simulink model "communication_codegen_check"  (R2024b)
settings: Solver=FixedStepDiscrete  StartTime=0.0  StopTime=0.1  FixedStep=0.001  RelTol=1e-3
settings Model: Creator=Administrator  LastModifiedBy=Administrator
settings OptimizationCC: EnhancedBackFolding=on  PassReuseOutputArgsAs=Individual arguments  ZeroExternalMemoryAtStartup=off  ZeroInternalMemoryAtStartup=off  MaxStackSize=64  OptimizeBlockOrder=speed  DifferentSizesBufferReuse=on  OptimizationCustomize=off  EfficientTunableParamExpr=on
settings DebuggingCC: ParameterTunabilityLossMsg=error
settings HardwareCC: ProdBitPerLong=64  ProdHWDeviceType=Intel->x86-64 (Linux 64)
settings SFSimCC: MATLABDynamicMemAlloc=off
settings RTWCC: Description=Embedded Coder  SystemTargetFile=ert.tlc  HardwareBoard=SimRT  TLCOptions="-aInlineSetEventsForThisBaseRateFcn=TLC_FALSE -aSuppressMultiTaskScheduler=TLC_FALSE  -aRateBasedStepFcn=0"  TemplateMakefile=ert_default_tmf  Toolchain=X280 portable-linux-toolchain
settings CodeAppCC: ForceParamTrailComments=on  IgnoreCustomStorageClasses=off  OperatorAnnotations=on  SimulinkDataObjDesc=on  SFDataObjDesc=on  InsertBlockDesc=on
settings ERTTargetCC: ExtMode=on  ExtModeTransport=2  ExtModeStaticAlloc=on  ExtModeMexFile=ext_xcp  ExtModeIntrfLevel=Level2 - Open  InlinedParameterPlacement=Hierarchical

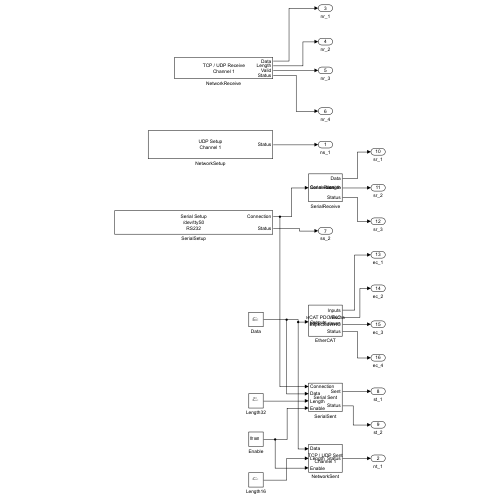
[thumbnail: Simulink's stored preview of the top-level diagram]
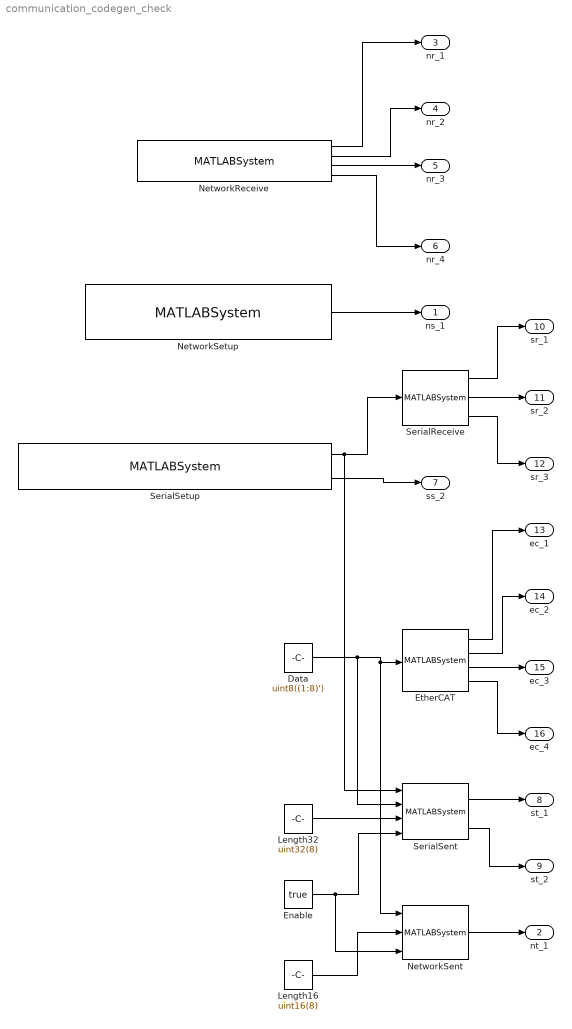
== system communication_codegen_check ==
  Data : Constant  Value=uint8((1:8)')
  Enable : Constant  Value=true
  EtherCAT : MATLABSystem  System=x280linux.ethercat.EtherCATExchange  Interface=eth1  ExpectedSlaves=1  OutputBytes=8  InputBytes=8  ReceiveTimeoutUs=500  SampleTime=0.001
      mask Type: x280linux.ethercat.EtherCATExchange
      mask Display:
      | disp(['EtherCAT PDO Exchange' char(10) 'eth1 / 1 slaves']);
      | port_label('input',1,'Outputs');
      | port_label('output',1,'Inputs');
      | port_label('output',2,'WKC');
      | port_label('output',3,'ExpectedWKC');
      | port_label('output',4,'Status');
  Length16 : Constant  Value=uint16(8)
  Length32 : Constant  Value=uint32(8)
  NetworkReceive : MATLABSystem  System=x280linux.net.TCPReceive  Channel=1  BufferSize=8  SampleTime=0.001
      mask Type: x280linux.net.TCPReceive
      mask Display:
      | disp(['TCP / UDP Receive' char(10) 'Channel 1']);
      | port_label('output',1,'Data');
      | port_label('output',2,'Length');
      | port_label('output',3,'Valid');
      | port_label('output',4,'Status');
  NetworkSent : MATLABSystem  System=x280linux.net.TCPSent  Channel=1
      mask Type: x280linux.net.TCPSent
      mask Display:
      | disp(['TCP / UDP Sent' char(10) 'Channel 1']);
      | port_label('input',1,'Data');
      | port_label('input',2,'Length');
      | port_label('input',3,'Enable');
      | port_label('output',1,'Status');
  NetworkSetup : MATLABSystem  System=x280linux.net.TCPSetup  Channel=1  Protocol=UDP  Role=Client  LocalAddress=0.0.0.0  LocalPort=45190  RemoteAddress=127.0.0.1  RemotePort=45191  SampleTime=0.001
      mask Type: x280linux.net.TCPSetup
      mask Display:
      | disp(['UDP Setup' char(10) 'Channel 1']);
      | port_label('output',1,'Status');
  SerialReceive : MATLABSystem  System=x280linux.serial.SerialReceive  BufferSize=8
      mask Type: x280linux.serial.SerialReceive
      mask Display:
      | disp('Serial Receive');
      | port_label('input',1,'Connection');
      | port_label('output',1,'Data');
      | port_label('output',2,'Length');
      | port_label('output',3,'Status');
  SerialSent : MATLABSystem  System=x280linux.serial.SerialSent
      mask Type: x280linux.serial.SerialSent
      mask Display:
      | disp('Serial Sent');
      | port_label('input',1,'Connection');
      | port_label('input',2,'Data');
      | port_label('input',3,'Length');
      | port_label('input',4,'Enable');
      | port_label('output',1,'Sent');
      | port_label('output',2,'Status');
  SerialSetup : MATLABSystem  System=x280linux.serial.SerialSetup  Device=/dev/ttyS0  BaudRate=115200  DataBits=8  Parity=None  StopBits=1  Mode=RS232  RS485Direction=Hardware auto  RTSOnSend=true  DelayBeforeSendMs=0  DelayAfterSendMs=0  SampleTime=0.001
      mask Type: x280linux.serial.SerialSetup
      mask Display:
      | disp(['Serial Setup' char(10) '/dev/ttyS0' char(10) 'RS232']);
      | port_label('output',1,'Connection');
      | port_label('output',2,'Status');
  ns_1 : Outport
  nt_1 : Outport  Port=2
  nr_1 : Outport  Port=3
  nr_2 : Outport  Port=4
  nr_3 : Outport  Port=5
  nr_4 : Outport  Port=6
  ss_2 : Outport  Port=7
  st_1 : Outport  Port=8
  st_2 : Outport  Port=9
  sr_1 : Outport  Port=10
  sr_2 : Outport  Port=11
  sr_3 : Outport  Port=12
  ec_1 : Outport  Port=13
  ec_2 : Outport  Port=14
  ec_3 : Outport  Port=15
  ec_4 : Outport  Port=16
  wires:
  EtherCAT/4 -> ec_4/1
  EtherCAT/3 -> ec_3/1
  EtherCAT/2 -> ec_2/1
  EtherCAT/1 -> ec_1/1
  SerialReceive/3 -> sr_3/1
  SerialReceive/2 -> sr_2/1
  SerialReceive/1 -> sr_1/1
  SerialSent/2 -> st_2/1
  SerialSent/1 -> st_1/1
  SerialSetup/2 -> ss_2/1
  NetworkReceive/4 -> nr_4/1
  NetworkReceive/3 -> nr_3/1
  NetworkReceive/2 -> nr_2/1
  NetworkReceive/1 -> nr_1/1
  NetworkSent/1 -> nt_1/1
  NetworkSetup/1 -> ns_1/1
  Length32/1 -> SerialSent/3
  SerialSetup/1 -> SerialSent/1, SerialReceive/1
  Enable/1 -> NetworkSent/3, SerialSent/4
  Length16/1 -> NetworkSent/2
  Data/1 -> NetworkSent/1, EtherCAT/1, SerialSent/2
